simulink model "BMS_MIL"  (R2025b)
settings: Solver=FixedStepAuto  StartTime=0.0  StopTime=360  FixedStep=Ts  RelTol=1e-3
InitFcn:
  | init_BMS
undefined symbols (not defined in the file): Ts
libraries: BMS_Library x2
settings Model: Creator=Khadija  LastModifiedBy=Khadija

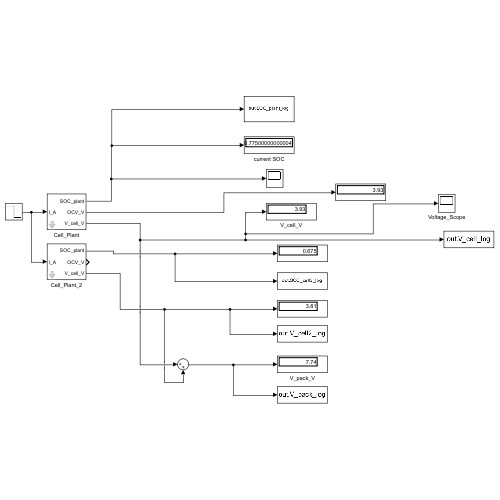
[thumbnail: Simulink's stored preview of the top-level diagram]
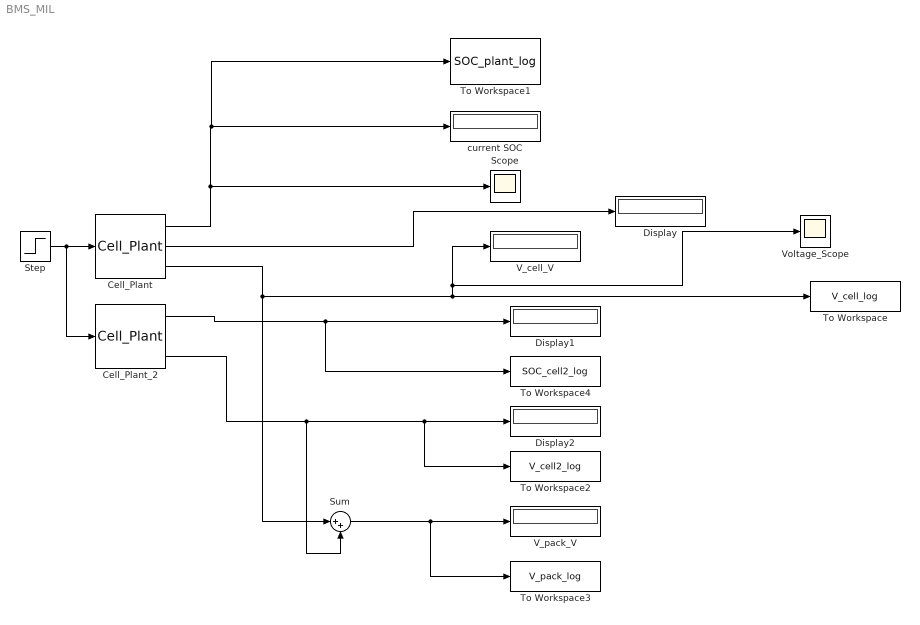
== system BMS_MIL ==
  Cell_Plant : BMS_Library/Cell_Plant  SOC_init=SOC0_plant
  Cell_Plant_2 : BMS_Library/Cell_Plant  SOC_init=SOC0_cell2
  Display : Display
  Display1 : Display
  Display2 : Display
  Scope : Scope
      settings: ActiveDisplayYMinimum=0.772169295711346  ActiveDisplayYMaximum=0.77569370148712624
  Step : Step  Time=180  Before=1  After=0  SampleTime=Ts
  Sum : Sum  Inputs=|++
  To Workspace : ToWorkspace  VariableName=V_cell_log  SaveFormat=Timeseries  SampleTime=-1
  To Workspace1 : ToWorkspace  VariableName=SOC_plant_log  SaveFormat=Timeseries  SampleTime=-1
  To Workspace2 : ToWorkspace  VariableName=V_cell2_log  SaveFormat=Timeseries  SampleTime=-1
  To Workspace3 : ToWorkspace  VariableName=V_pack_log  SaveFormat=Timeseries  SampleTime=-1
  To Workspace4 : ToWorkspace  VariableName=SOC_cell2_log  SaveFormat=Timeseries  SampleTime=-1
  V_cell_V : Display
  V_pack_V : Display
  Voltage_Scope : Scope
      settings: ActiveDisplayYMinimum=3.880451259553837  ActiveDisplayYMaximum=3.9932322443788055
  current SOC : Display
  wires:
  Cell_Plant/1 -> Scope/1, To Workspace1/1, current SOC/1
  Cell_Plant/2 -> Display/1
  Cell_Plant/3 -> To Workspace/1, Voltage_Scope/1, V_cell_V/1, Sum/1
  Step/1 -> Cell_Plant_2/1, Cell_Plant/1
  Cell_Plant_2/3 -> Sum/2, To Workspace2/1, Display2/1
  Sum/1 -> To Workspace3/1, V_pack_V/1
  Cell_Plant_2/1 -> To Workspace4/1, Display1/1
